simulink model "LQR_CTV_Tuning"  (R2026b)
settings: Solver=VariableStepAuto
undefined symbols (not defined in the file): ctrl_ts_in, ctrl_ts_out, K1flat_ctv, K2grid_ctv, Target_Trajectory, tgrid, unom
settings Model: Creator=asing  LastModifiedBy=asing

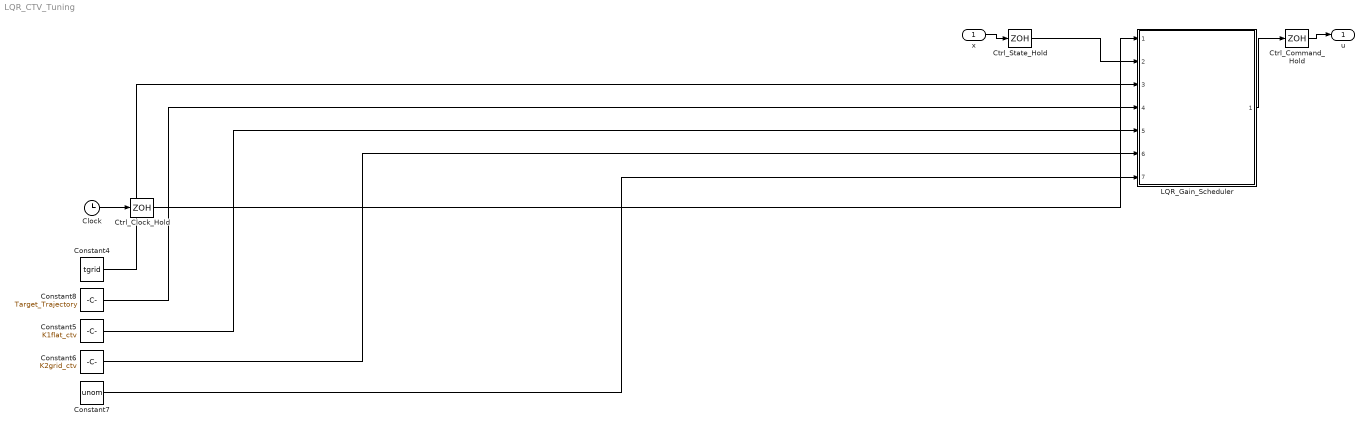
== system LQR_CTV_Tuning ==
  x : Inport
  Clock : Clock
  Constant4 : Constant  Value=tgrid
  Constant5 : Constant  Value=K1flat_ctv
  Constant6 : Constant  Value=K2grid_ctv
  Constant7 : Constant  Value=unom
  Constant8 : Constant  Value=Target_Trajectory
  Ctrl_Clock_Hold : ZeroOrderHold  SampleTime=ctrl_ts_in
  Ctrl_Command_Hold : ZeroOrderHold  SampleTime=ctrl_ts_out
  Ctrl_State_Hold : ZeroOrderHold  SampleTime=ctrl_ts_in
  LQR_Gain_Scheduler : Subsystem  ReferencedSubsystem=LQR_Gain_Scheduler
  u : Outport
  wires:
  Constant7/1 -> LQR_Gain_Scheduler/7
  Constant6/1 -> LQR_Gain_Scheduler/6
  Constant5/1 -> LQR_Gain_Scheduler/5
  Constant8/1 -> LQR_Gain_Scheduler/4
  Constant4/1 -> LQR_Gain_Scheduler/3
  x/1 -> Ctrl_State_Hold/1
  Ctrl_State_Hold/1 -> LQR_Gain_Scheduler/2
  Clock/1 -> Ctrl_Clock_Hold/1
  Ctrl_Clock_Hold/1 -> LQR_Gain_Scheduler/1
  LQR_Gain_Scheduler/1 -> Ctrl_Command_Hold/1
  Ctrl_Command_Hold/1 -> u/1
